simulink library "tip_assist_lib"  (Simulink 9.0)
settings: Solver=VariableStepAuto  StartTime=0.0  StopTime=10.0  RelTol=1e-3
settings Model: Creator=currisd  LastModifiedBy=currisd

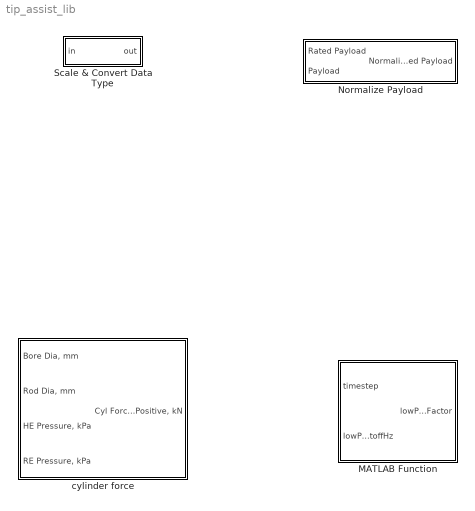
== system tip_assist_lib ==
  MATLAB Function : MATLAB Function  TreatAsAtomicUnit=on
  Normalize Payload : Subsystem
  Scale & Convert Data Type : Subsystem  mask{scaling=1}
      mask prompts: scaling "Scaling Factor"
      mask Display: disp(num2str(scaling))
  cylinder force : Subsystem

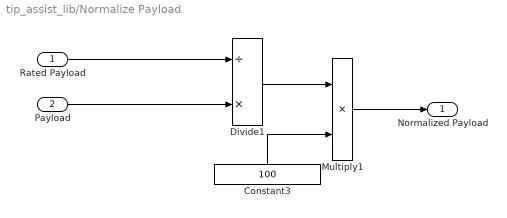
== system tip_assist_lib/Normalize Payload ==
  Rated Payload : Inport
  Payload : Inport  Port=2
  Constant3 : Constant  Value=100  OutDataTypeStr=single  SampleTime=-1
  Divide1 : Product  Inputs=/*
  Multiply1 : Product  SaturateOnIntegerOverflow=on  RndMeth=Zero  InputSameDT=on  OutDataTypeStr=Inherit: Same as first input
  " Normalized Payload" : Outport
  wires:
  Multiply1/1 -> " Normalized Payload"/1
  Constant3/1 -> Multiply1/2
  Rated Payload/1 -> Divide1/1
  Payload/1 -> Divide1/2
  Divide1/1 -> Multiply1/1

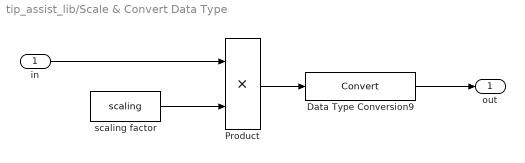
== system tip_assist_lib/Scale & Convert Data Type ==
  in : Inport
  Data Type Conversion9 : DataTypeConversion  RndMeth=Nearest  SaturateOnIntegerOverflow=on
  Product : Product
  scaling factor : Constant  Value=scaling  SampleTime=-1
  out : Outport
  wires:
  Product/1 -> Data Type Conversion9/1
  scaling factor/1 -> Product/2
  Data Type Conversion9/1 -> out/1
  in/1 -> Product/1

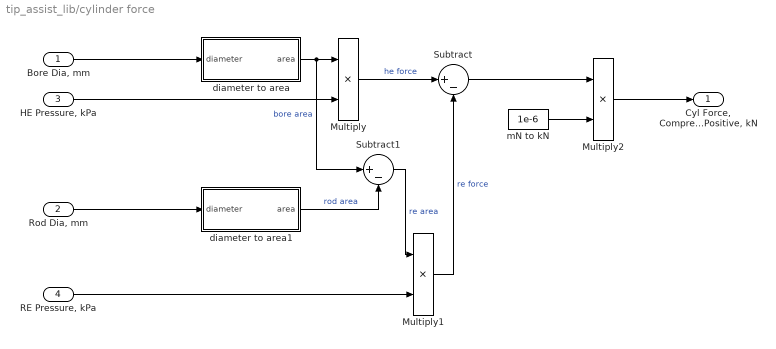
== system tip_assist_lib/cylinder force ==
  "Bore Dia, mm" : Inport
  "Rod Dia, mm" : Inport  Port=2
  "HE Pressure, kPa" : Inport  Port=3
  "RE Pressure, kPa" : Inport  Port=4
  Multiply : Product  SaturateOnIntegerOverflow=on  RndMeth=Zero  InputSameDT=on  OutDataTypeStr=Inherit: Same as first input
  Multiply1 : Product  SaturateOnIntegerOverflow=on  RndMeth=Zero  InputSameDT=on  OutDataTypeStr=Inherit: Same as first input
  Multiply2 : Product  SaturateOnIntegerOverflow=on  RndMeth=Zero  InputSameDT=on  OutDataTypeStr=Inherit: Same as first input
  Subtract : Sum  Inputs=|+-  SaturateOnIntegerOverflow=on  InputSameDT=on  OutDataTypeStr=Inherit: Same as first input
  Subtract1 : Sum  Inputs=|+-  SaturateOnIntegerOverflow=on  InputSameDT=on  OutDataTypeStr=Inherit: Same as first input
  diameter to area : Subsystem
  diameter to area1 : Subsystem
  mN to kN : Constant  Value=1e-6  OutDataTypeStr=single
  "Cyl Force, Compression Positive, kN" : Outport
  wires:
  Multiply2/1 -> "Cyl Force, Compression Positive, kN"/1
  mN to kN/1 -> Multiply2/2
  Subtract1/1 -> Multiply1/1  "re area"
  "Rod Dia, mm"/1 -> diameter to area1/1(diameter)
  "RE Pressure, kPa"/1 -> Multiply1/2
  diameter to area1/1(area) -> Subtract1/2  "rod area"
  diameter to area/1(area) -> Multiply/1, Subtract1/1  "bore area"
  Multiply/1 -> Subtract/1  "he force"
  Multiply1/1 -> Subtract/2  "re force"
  "Bore Dia, mm"/1 -> diameter to area/1(diameter)
  Subtract/1 -> Multiply2/1
  "HE Pressure, kPa"/1 -> Multiply/2

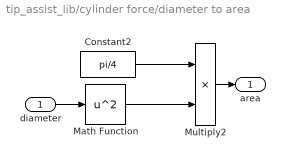
== system tip_assist_lib/cylinder force/diameter to area ==
  diameter : Inport
  Constant2 : Constant  Value=pi/4  OutDataTypeStr=single
  Math Function : Math  Operator=square  OutputSignalType=real  SaturateOnIntegerOverflow=on
  Multiply2 : Product  SaturateOnIntegerOverflow=on  RndMeth=Zero  InputSameDT=on  OutDataTypeStr=Inherit: Same as first input
  area : Outport
  wires:
  diameter/1 -> Math Function/1
  Multiply2/1 -> area/1
  Math Function/1 -> Multiply2/2
  Constant2/1 -> Multiply2/1

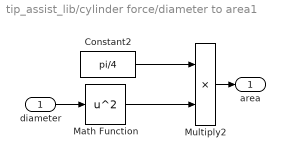
== system tip_assist_lib/cylinder force/diameter to area1 ==
  diameter : Inport
  Constant2 : Constant  Value=pi/4  OutDataTypeStr=single
  Math Function : Math  Operator=square  OutputSignalType=real  SaturateOnIntegerOverflow=on
  Multiply2 : Product  SaturateOnIntegerOverflow=on  RndMeth=Zero  InputSameDT=on  OutDataTypeStr=Inherit: Same as first input
  area : Outport
  wires:
  diameter/1 -> Math Function/1
  Multiply2/1 -> area/1
  Math Function/1 -> Multiply2/2
  Constant2/1 -> Multiply2/1

== matlab function MATLAB Function ==
  data: timestep input double; lowPassFilterFactor output double; lowPassFilterCutoffHz input double
function lowPassFilterFactor = calcFilterFactor(timestep, lowPassFilterCutoffHz)

% Low-pass filter cutoff (rad/s)
cutoff = lowPassFilterCutoffHz * (2 * pi);
% Low-pass filter angle (rad)
angle = cutoff * timestep;
% Filter factor corresponding to cutoff
lowPassFilterFactor = ...
    (cos(angle) - 1) + sqrt((cos(angle) - 3) * (cos(angle) - 1));
